simulink subsystem "Create3x3Matrix"  (R2024b)
settings: Solver=VariableStepAuto  StartTime=0.0  StopTime=10.0  RelTol=1e-3
settings Model: Creator=pierb  LastModifiedBy=pierb

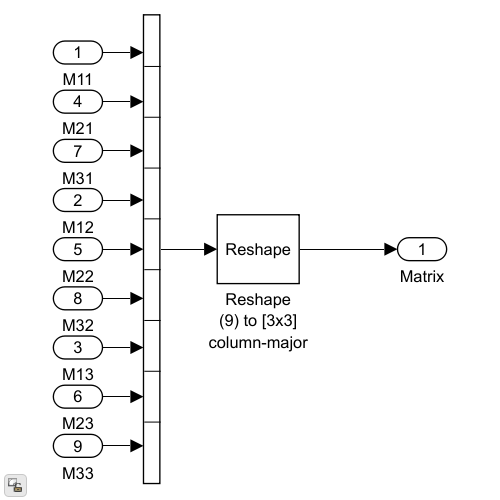
[thumbnail: Simulink's stored preview of the top-level diagram]
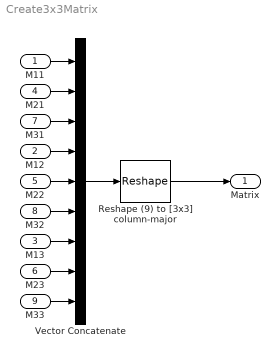
== system Create3x3Matrix ==
  M11 : Inport  PortDimensions=1
  M12 : Inport  Port=2  PortDimensions=1
  M13 : Inport  Port=3  PortDimensions=1
  M21 : Inport  Port=4  PortDimensions=1
  M22 : Inport  Port=5  PortDimensions=1
  M23 : Inport  Port=6  PortDimensions=1
  M31 : Inport  Port=7  PortDimensions=1
  M32 : Inport  Port=8  PortDimensions=1
  M33 : Inport  Port=9  PortDimensions=1
  Reshape (9) to [3x3] column-major : Reshape  OutputDimensionality=Customize  OutputDimensions=[3,3]
  Vector Concatenate : Concatenate  NumInputs=9
  Matrix : Outport  PortDimensions=[3 3]  VectorParamsAs1DForOutWhenUnconnected=off
  wires:
  Vector Concatenate/1 -> Reshape (9) to [3x3] column-major/1
  M21/1 -> Vector Concatenate/2
  M13/1 -> Vector Concatenate/7
  M22/1 -> Vector Concatenate/5
  M23/1 -> Vector Concatenate/8
  M31/1 -> Vector Concatenate/3
  M33/1 -> Vector Concatenate/9
  Reshape (9) to [3x3] column-major/1 -> Matrix/1
  M11/1 -> Vector Concatenate/1
  M12/1 -> Vector Concatenate/4
  M32/1 -> Vector Concatenate/6
